simulink model "fixed_point_model"  (R2022b)
settings: Solver=FixedStepDiscrete  StartTime=0.0  StopTime=0.01  FixedStep=1e-10  RelTol=1e-3
undefined symbols (not defined in the file or in its folder): theta_input
libraries: dspsigops x206, dspsrcs4 x16, simulink x8, commdigbbndpm3 x1, commrandsrc3 x1
(part 5 of 6)

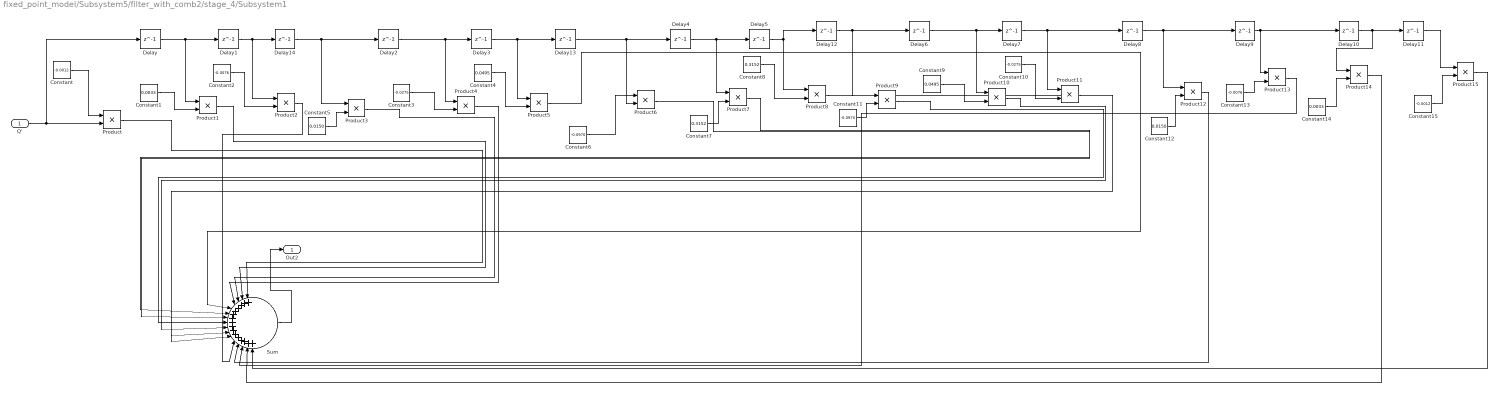
== system fixed_point_model/Subsystem5/filter_with_comb2/stage_4/Subsystem1 ==
  Q' : Inport
  Constant : Constant  Value=-0.0012
  Constant1 : Constant  Value=0.0033
  Constant10 : Constant  Value=-0.0275
  Constant11 : Constant  Value=-0.0970
  Constant12 : Constant  Value=0.0150
  Constant13 : Constant  Value=-0.0076
  Constant14 : Constant  Value=0.0033
  Constant15 : Constant  Value=-0.0012
  Constant2 : Constant  Value=-0.0076
  Constant3 : Constant  Value=-0.0275
  Constant4 : Constant  Value=0.0495
  Constant5 : Constant  Value=0.0150
  Constant6 : Constant  Value=-0.0970
  Constant7 : Constant  Value=0.3152
  Constant8 : Constant  Value=0.3152
  Constant9 : Constant  Value=0.0495
  Delay{,1..14} (15 alike) : Delay  DelayLength=1  InitialCondition=0  InputProcessing=Columns as channels (frame based)
  Product{,1..15} (16 alike) : Product
  Sum : Sum  Inputs=|++++++++++++++++
  Out2 : Outport
  wires:
  Constant1/1 -> Product1/2
  Delay2/1 -> Delay3/1, Product4/1
  Constant10/1 -> Product11/2
  Constant9/1 -> Product10/2
  Delay/1 -> Delay1/1, Product1/1
  Delay4/1 -> Delay5/1, Product7/1
  Constant3/1 -> Product4/2
  Product8/1 -> Sum/11
  Product6/1 -> Sum/6
  Delay1/1 -> Product2/1, Delay14/1
  Delay5/1 -> Delay12/1, Product8/1
  Constant8/1 -> Product8/2
  Q'/1 -> Delay/1, Product/2
  Delay6/1 -> Delay7/1, Product10/1
  Constant/1 -> Product/1
  Constant11/1 -> Product9/2
  Product10/1 -> Sum/9
  Delay7/1 -> Delay8/1, Product11/1
  Product9/1 -> Sum/8
  Delay3/1 -> Product5/1, Delay13/1
  Constant4/1 -> Product5/2
  Product3/1 -> Sum/3
  Product5/1 -> Sum/5
  Constant2/1 -> Product2/2
  Constant5/1 -> Product3/2
  Constant7/1 -> Product7/2
  Product11/1 -> Sum/10
  Constant6/1 -> Product6/1
  Product/1 -> Sum/1
  Product1/1 -> Sum/2
  Product7/1 -> Sum/7
  Product4/1 -> Sum/4
  Sum/1 -> Out2/1
  Product2/1 -> Sum/12
  Constant12/1 -> Product12/2
  Delay8/1 -> Product12/1, Delay9/1
  Constant13/1 -> Product13/2
  Delay9/1 -> Delay10/1, Product13/1
  Constant14/1 -> Product14/2
  Delay10/1 -> Delay11/1, Product14/1
  Delay11/1 -> Product15/1
  Constant15/1 -> Product15/2
  Product12/1 -> Sum/13
  Product13/1 -> Sum/14
  Product14/1 -> Sum/15
  Product15/1 -> Sum/16
  Delay12/1 -> Delay6/1, Product9/1
  Delay13/1 -> Delay4/1, Product6/2
  Delay14/1 -> Delay2/1, Product3/1

== system fixed_point_model/Subsystem6/filter_with_comb1/Stage_1/Subsystem ==
  In1 : Inport
  Constant : Constant
  Constant1 : Constant  Value=42
  Constant2 : Constant  Value=21
  Delay1 : Delay  DelayLength=1  InitialCondition=0  InputProcessing=Columns as channels (frame based)
  Delay2 : Delay  DelayLength=1  InitialCondition=0  InputProcessing=Columns as channels (frame based)
  Product : Product
  Product1 : Product
  Product2 : Product
  Sum : Sum  Inputs=|+++
  Out1 : Outport
  wires:
  Constant1/1 -> Product1/2
  In1/1 -> Product/1, Delay1/1
  Product1/1 -> Sum/2
  Product/1 -> Sum/1
  Sum/1 -> Out1/1
  Constant/1 -> Product/2
  Delay1/1 -> Delay2/1, Product1/1
  Delay2/1 -> Product2/1
  Constant2/1 -> Product2/2
  Product2/1 -> Sum/3

== system fixed_point_model/Subsystem6/filter_with_comb1/Stage_1/Subsystem1 ==
  In2 : Inport
  Constant2 : Constant  Value=3
  Constant3 : Constant  Value=46
  Constant4 : Constant  Value=15
  Delay2 : Delay  DelayLength=1  InitialCondition=0  InputProcessing=Columns as channels (frame based)
  Delay3 : Delay  DelayLength=1  InitialCondition=0  InputProcessing=Columns as channels (frame based)
  Product2 : Product
  Product3 : Product
  Product4 : Product
  Sum1 : Sum  Inputs=|+++
  Out2 : Outport
  wires:
  Delay3/1 -> Product4/1
  Delay2/1 -> Delay3/1, Product3/1
  Sum1/1 -> Out2/1
  Constant2/1 -> Product2/2
  Product2/1 -> Sum1/1
  Constant3/1 -> Product3/2
  Product3/1 -> Sum1/2
  Constant4/1 -> Product4/2
  In2/1 -> Delay2/1, Product2/1
  Product4/1 -> Sum1/3

== system fixed_point_model/Subsystem6/filter_with_comb1/Stage_1/Subsystem2 ==
  In2 : Inport
  Constant2 : Constant  Value=6
  Constant3 : Constant  Value=48
  Constant4 : Constant  Value=10
  Delay2 : Delay  DelayLength=1  InitialCondition=0  InputProcessing=Columns as channels (frame based)
  Delay3 : Delay  DelayLength=1  InitialCondition=0  InputProcessing=Columns as channels (frame based)
  Product2 : Product
  Product3 : Product
  Product4 : Product
  Sum1 : Sum  Inputs=|+++
  Out2 : Outport
  wires:
  In2/1 -> Delay2/1, Product2/1
  Constant4/1 -> Product4/2
  Product2/1 -> Sum1/1
  Constant3/1 -> Product3/2
  Constant2/1 -> Product2/2
  Delay2/1 -> Delay3/1, Product3/1
  Product3/1 -> Sum1/2
  Sum1/1 -> Out2/1
  Delay3/1 -> Product4/1
  Product4/1 -> Sum1/3

== system fixed_point_model/Subsystem6/filter_with_comb1/Stage_1/Subsystem3 ==
  In2 : Inport
  Constant2 : Constant  Value=10
  Constant3 : Constant  Value=48
  Constant4 : Constant  Value=6
  Delay2 : Delay  DelayLength=1  InitialCondition=0  InputProcessing=Columns as channels (frame based)
  Delay3 : Delay  DelayLength=1  InitialCondition=0  InputProcessing=Columns as channels (frame based)
  Product2 : Product
  Product3 : Product
  Product4 : Product
  Sum1 : Sum  Inputs=|+++
  Out2 : Outport
  wires:
  In2/1 -> Delay2/1, Product2/1
  Constant4/1 -> Product4/2
  Product2/1 -> Sum1/1
  Constant3/1 -> Product3/2
  Constant2/1 -> Product2/2
  Delay2/1 -> Delay3/1, Product3/1
  Product3/1 -> Sum1/2
  Sum1/1 -> Out2/1
  Delay3/1 -> Product4/1
  Product4/1 -> Sum1/3

== system fixed_point_model/Subsystem6/filter_with_comb1/Stage_1/Subsystem4 ==
  In2 : Inport
  Constant2 : Constant  Value=15
  Constant3 : Constant  Value=46
  Constant4 : Constant  Value=3
  Delay2 : Delay  DelayLength=1  InitialCondition=0
  Delay3 : Delay  DelayLength=1  InitialCondition=0  InputProcessing=Columns as channels (frame based)
  Product2 : Product
  Product3 : Product
  Product4 : Product
  Sum1 : Sum  Inputs=|+++++
  Out2 : Outport
  wires:
  In2/1 -> Delay2/1, Product2/1
  Product4/1 -> Sum1/4
  Constant4/1 -> Product4/2
  Product2/1 -> Sum1/1
  Constant3/1 -> Product3/2
  Constant2/1 -> Product2/2
  Delay2/1 -> Delay3/1, Product3/1
  Product3/1 -> Sum1/2
  Sum1/1 -> Out2/1
  Delay3/1 -> Product4/1

== system fixed_point_model/Subsystem6/filter_with_comb1/Stage_1/Subsystem5 ==
  In2 : Inport
  Constant2 : Constant  Value=21
  Constant3 : Constant  Value=42
  Constant4 : Constant
  Delay2 : Delay  DelayLength=1  InitialCondition=0  InputProcessing=Columns as channels (frame based)
  Delay3 : Delay  DelayLength=1  InitialCondition=0  InputProcessing=Columns as channels (frame based)
  Product2 : Product
  Product3 : Product
  Product4 : Product
  Sum1 : Sum  Inputs=|+++
  Out2 : Outport
  wires:
  In2/1 -> Delay2/1, Product2/1
  Constant4/1 -> Product4/2
  Product2/1 -> Sum1/1
  Constant3/1 -> Product3/2
  Constant2/1 -> Product2/2
  Delay2/1 -> Delay3/1, Product3/1
  Product3/1 -> Sum1/2
  Sum1/1 -> Out2/1
  Delay3/1 -> Product4/1
  Product4/1 -> Sum1/3

== system fixed_point_model/Subsystem6/filter_with_comb1/Stage_1/Subsystem6 ==
  In2 : Inport
  Constant2 : Constant  Value=28
  Constant3 : Constant  Value=36
  Delay2 : Delay  DelayLength=1  InitialCondition=0  InputProcessing=Columns as channels (frame based)
  Product2 : Product
  Product3 : Product
  Sum1 : Sum  Inputs=|++
  Out2 : Outport
  wires:
  In2/1 -> Delay2/1, Product2/1
  Product2/1 -> Sum1/1
  Constant3/1 -> Product3/2
  Constant2/1 -> Product2/2
  Delay2/1 -> Product3/1
  Product3/1 -> Sum1/2
  Sum1/1 -> Out2/1

== system fixed_point_model/Subsystem6/filter_with_comb1/Stage_1/Subsystem7 ==
  In2 : Inport
  Constant2 : Constant  Value=36
  Constant3 : Constant  Value=28
  Delay2 : Delay  DelayLength=1  InitialCondition=0  InputProcessing=Columns as channels (frame based)
  Product2 : Product
  Product3 : Product
  Sum1 : Sum  Inputs=|++
  Out2 : Outport
  wires:
  In2/1 -> Delay2/1, Product2/1
  Product2/1 -> Sum1/1
  Constant3/1 -> Product3/2
  Constant2/1 -> Product2/2
  Delay2/1 -> Product3/1
  Product3/1 -> Sum1/2
  Sum1/1 -> Out2/1

== system fixed_point_model/Subsystem6/filter_with_comb1/stage_3/Subsystem ==
  In1 : Inport
  Constant : Constant  Value=0.0006
  Constant1 : Constant  Value=-0.0051
  Constant2 : Constant  Value=0.0222
  Constant3 : Constant  Value=-0.0735
  Constant4 : Constant  Value=0.3058
  Constant5 : Constant  Value=0.3058
  Constant6 : Constant  Value=-0.0735
  Constant7 : Constant  Value=0.0222
  Constant8 : Constant  Value=-0.0051
  Constant9 : Constant  Value=0.0006
  Delay{1..9} (9 alike) : Delay  DelayLength=1  InitialCondition=0  InputProcessing=Columns as channels (frame based)
  Product{,1..9} (10 alike) : Product
  Sum : Sum  Inputs=|++++++++++
  Out1 : Outport
  wires:
  Product/1 -> Sum/1
  Product2/1 -> Sum/3
  Delay3/1 -> Product1/1, Delay4/1
  Sum/1 -> Out1/1
  Delay4/1 -> Product2/1, Delay5/1
  Product3/1 -> Sum/4
  In1/1 -> Product/2, Delay3/1
  Constant2/1 -> Product2/2
  Constant3/1 -> Product3/2
  Constant/1 -> Product/1
  Product1/1 -> Sum/2
  Constant1/1 -> Product1/2
  Delay5/1 -> Delay8/1, Product3/1
  Constant7/1 -> Product7/2
  Constant5/1 -> Product5/2
  Constant4/1 -> Product4/1
  Delay6/1 -> Product7/1, Delay9/1
  Delay2/1 -> Delay6/1, Product6/1
  Delay1/1 -> Delay2/1, Product5/1
  Constant6/1 -> Product6/2
  Constant8/1 -> Product8/2
  Constant9/1 -> Product9/2
  Delay7/1 -> Product9/1
  Product5/1 -> Sum/5
  Product6/1 -> Sum/6
  Product7/1 -> Sum/7
  Product8/1 -> Sum/8
  Product9/1 -> Sum/9
  Product4/1 -> Sum/10
  Delay8/1 -> Product4/2, Delay1/1
  Delay9/1 -> Product8/1, Delay7/1

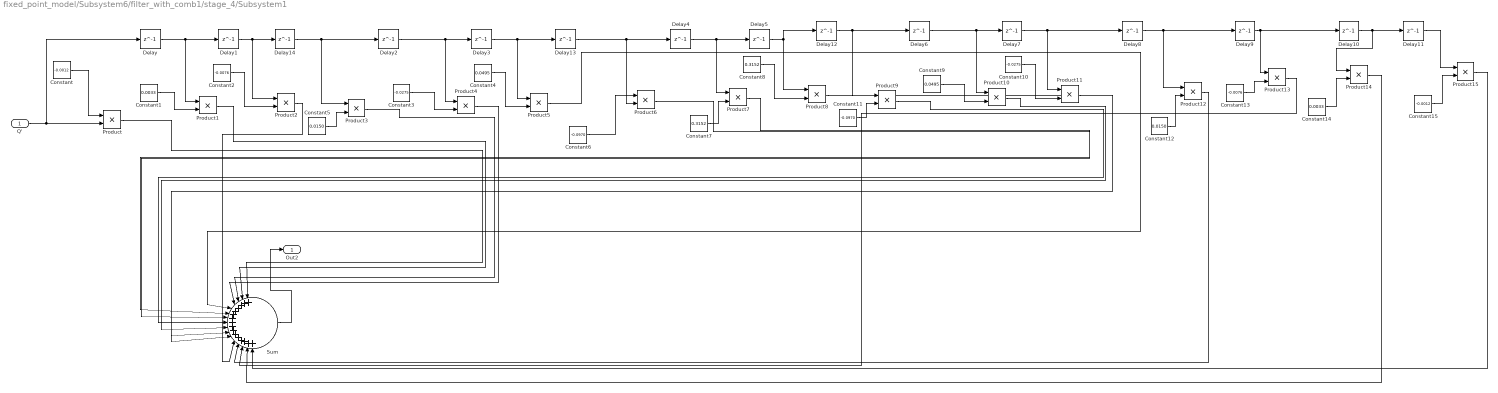
== system fixed_point_model/Subsystem6/filter_with_comb1/stage_4/Subsystem1 ==
  Q' : Inport
  Constant : Constant  Value=-0.0012
  Constant1 : Constant  Value=0.0033
  Constant10 : Constant  Value=-0.0275
  Constant11 : Constant  Value=-0.0970
  Constant12 : Constant  Value=0.0150
  Constant13 : Constant  Value=-0.0076
  Constant14 : Constant  Value=0.0033
  Constant15 : Constant  Value=-0.0012
  Constant2 : Constant  Value=-0.0076
  Constant3 : Constant  Value=-0.0275
  Constant4 : Constant  Value=0.0495
  Constant5 : Constant  Value=0.0150
  Constant6 : Constant  Value=-0.0970
  Constant7 : Constant  Value=0.3152
  Constant8 : Constant  Value=0.3152
  Constant9 : Constant  Value=0.0495
  Delay{,1..14} (15 alike) : Delay  DelayLength=1  InitialCondition=0  InputProcessing=Columns as channels (frame based)
  Product{,1..15} (16 alike) : Product
  Sum : Sum  Inputs=|++++++++++++++++
  Out2 : Outport
  wires:
  Constant1/1 -> Product1/2
  Delay2/1 -> Delay3/1, Product4/1
  Constant10/1 -> Product11/2
  Constant9/1 -> Product10/2
  Delay/1 -> Delay1/1, Product1/1
  Delay4/1 -> Delay5/1, Product7/1
  Constant3/1 -> Product4/2
  Product8/1 -> Sum/11
  Product6/1 -> Sum/6
  Delay1/1 -> Product2/1, Delay14/1
  Delay5/1 -> Delay12/1, Product8/1
  Constant8/1 -> Product8/2
  Q'/1 -> Delay/1, Product/2
  Delay6/1 -> Delay7/1, Product10/1
  Constant/1 -> Product/1
  Constant11/1 -> Product9/2
  Product10/1 -> Sum/9
  Delay7/1 -> Delay8/1, Product11/1
  Product9/1 -> Sum/8
  Delay3/1 -> Product5/1, Delay13/1
  Constant4/1 -> Product5/2
  Product3/1 -> Sum/3
  Product5/1 -> Sum/5
  Constant2/1 -> Product2/2
  Constant5/1 -> Product3/2
  Constant7/1 -> Product7/2
  Product11/1 -> Sum/10
  Constant6/1 -> Product6/1
  Product/1 -> Sum/1
  Product1/1 -> Sum/2
  Product7/1 -> Sum/7
  Product4/1 -> Sum/4
  Sum/1 -> Out2/1
  Product2/1 -> Sum/12
  Constant12/1 -> Product12/2
  Delay8/1 -> Product12/1, Delay9/1
  Constant13/1 -> Product13/2
  Delay9/1 -> Delay10/1, Product13/1
  Constant14/1 -> Product14/2
  Delay10/1 -> Delay11/1, Product14/1
  Delay11/1 -> Product15/1
  Constant15/1 -> Product15/2
  Product12/1 -> Sum/13
  Product13/1 -> Sum/14
  Product14/1 -> Sum/15
  Product15/1 -> Sum/16
  Delay12/1 -> Delay6/1, Product9/1
  Delay13/1 -> Delay4/1, Product6/2
  Delay14/1 -> Delay2/1, Product3/1

== system fixed_point_model/Subsystem6/filter_with_comb2/Stage_1/Subsystem ==
  In1 : Inport
  Constant : Constant
  Constant1 : Constant  Value=42
  Constant2 : Constant  Value=21
  Delay1 : Delay  DelayLength=1  InitialCondition=0  InputProcessing=Columns as channels (frame based)
  Delay2 : Delay  DelayLength=1  InitialCondition=0  InputProcessing=Columns as channels (frame based)
  Product : Product
  Product1 : Product
  Product2 : Product
  Sum : Sum  Inputs=|+++
  Out1 : Outport
  wires:
  Constant1/1 -> Product1/2
  In1/1 -> Product/1, Delay1/1
  Product1/1 -> Sum/2
  Product/1 -> Sum/1
  Sum/1 -> Out1/1
  Constant/1 -> Product/2
  Delay1/1 -> Delay2/1, Product1/1
  Delay2/1 -> Product2/1
  Constant2/1 -> Product2/2
  Product2/1 -> Sum/3

== system fixed_point_model/Subsystem6/filter_with_comb2/Stage_1/Subsystem1 ==
  In2 : Inport
  Constant2 : Constant  Value=3
  Constant3 : Constant  Value=46
  Constant4 : Constant  Value=15
  Delay2 : Delay  DelayLength=1  InitialCondition=0  InputProcessing=Columns as channels (frame based)
  Delay3 : Delay  DelayLength=1  InitialCondition=0  InputProcessing=Columns as channels (frame based)
  Product2 : Product
  Product3 : Product
  Product4 : Product
  Sum1 : Sum  Inputs=|+++
  Out2 : Outport
  wires:
  Delay3/1 -> Product4/1
  Delay2/1 -> Delay3/1, Product3/1
  Sum1/1 -> Out2/1
  Constant2/1 -> Product2/2
  Product2/1 -> Sum1/1
  Constant3/1 -> Product3/2
  Product3/1 -> Sum1/2
  Constant4/1 -> Product4/2
  In2/1 -> Delay2/1, Product2/1
  Product4/1 -> Sum1/3

== system fixed_point_model/Subsystem6/filter_with_comb2/Stage_1/Subsystem2 ==
  In2 : Inport
  Constant2 : Constant  Value=6
  Constant3 : Constant  Value=48
  Constant4 : Constant  Value=10
  Delay2 : Delay  DelayLength=1  InitialCondition=0  InputProcessing=Columns as channels (frame based)
  Delay3 : Delay  DelayLength=1  InitialCondition=0  InputProcessing=Columns as channels (frame based)
  Product2 : Product
  Product3 : Product
  Product4 : Product
  Sum1 : Sum  Inputs=|+++
  Out2 : Outport
  wires:
  In2/1 -> Delay2/1, Product2/1
  Constant4/1 -> Product4/2
  Product2/1 -> Sum1/1
  Constant3/1 -> Product3/2
  Constant2/1 -> Product2/2
  Delay2/1 -> Delay3/1, Product3/1
  Product3/1 -> Sum1/2
  Sum1/1 -> Out2/1
  Delay3/1 -> Product4/1
  Product4/1 -> Sum1/3

== system fixed_point_model/Subsystem6/filter_with_comb2/Stage_1/Subsystem3 ==
  In2 : Inport
  Constant2 : Constant  Value=10
  Constant3 : Constant  Value=48
  Constant4 : Constant  Value=6
  Delay2 : Delay  DelayLength=1  InitialCondition=0  InputProcessing=Columns as channels (frame based)
  Delay3 : Delay  DelayLength=1  InitialCondition=0  InputProcessing=Columns as channels (frame based)
  Product2 : Product
  Product3 : Product
  Product4 : Product
  Sum1 : Sum  Inputs=|+++
  Out2 : Outport
  wires:
  In2/1 -> Delay2/1, Product2/1
  Constant4/1 -> Product4/2
  Product2/1 -> Sum1/1
  Constant3/1 -> Product3/2
  Constant2/1 -> Product2/2
  Delay2/1 -> Delay3/1, Product3/1
  Product3/1 -> Sum1/2
  Sum1/1 -> Out2/1
  Delay3/1 -> Product4/1
  Product4/1 -> Sum1/3

== system fixed_point_model/Subsystem6/filter_with_comb2/Stage_1/Subsystem4 ==
  In2 : Inport
  Constant2 : Constant  Value=15
  Constant3 : Constant  Value=46
  Constant4 : Constant  Value=3
  Delay2 : Delay  DelayLength=1  InitialCondition=0
  Delay3 : Delay  DelayLength=1  InitialCondition=0  InputProcessing=Columns as channels (frame based)
  Product2 : Product
  Product3 : Product
  Product4 : Product
  Sum1 : Sum  Inputs=|+++++
  Out2 : Outport
  wires:
  In2/1 -> Delay2/1, Product2/1
  Product4/1 -> Sum1/4
  Constant4/1 -> Product4/2
  Product2/1 -> Sum1/1
  Constant3/1 -> Product3/2
  Constant2/1 -> Product2/2
  Delay2/1 -> Delay3/1, Product3/1
  Product3/1 -> Sum1/2
  Sum1/1 -> Out2/1
  Delay3/1 -> Product4/1

== system fixed_point_model/Subsystem6/filter_with_comb2/Stage_1/Subsystem5 ==
  In2 : Inport
  Constant2 : Constant  Value=21
  Constant3 : Constant  Value=42
  Constant4 : Constant
  Delay2 : Delay  DelayLength=1  InitialCondition=0  InputProcessing=Columns as channels (frame based)
  Delay3 : Delay  DelayLength=1  InitialCondition=0  InputProcessing=Columns as channels (frame based)
  Product2 : Product
  Product3 : Product
  Product4 : Product
  Sum1 : Sum  Inputs=|+++
  Out2 : Outport
  wires:
  In2/1 -> Delay2/1, Product2/1
  Constant4/1 -> Product4/2
  Product2/1 -> Sum1/1
  Constant3/1 -> Product3/2
  Constant2/1 -> Product2/2
  Delay2/1 -> Delay3/1, Product3/1
  Product3/1 -> Sum1/2
  Sum1/1 -> Out2/1
  Delay3/1 -> Product4/1
  Product4/1 -> Sum1/3

== system fixed_point_model/Subsystem6/filter_with_comb2/Stage_1/Subsystem6 ==
  In2 : Inport
  Constant2 : Constant  Value=28
  Constant3 : Constant  Value=36
  Delay2 : Delay  DelayLength=1  InitialCondition=0  InputProcessing=Columns as channels (frame based)
  Product2 : Product
  Product3 : Product
  Sum1 : Sum  Inputs=|++
  Out2 : Outport
  wires:
  In2/1 -> Delay2/1, Product2/1
  Product2/1 -> Sum1/1
  Constant3/1 -> Product3/2
  Constant2/1 -> Product2/2
  Delay2/1 -> Product3/1
  Product3/1 -> Sum1/2
  Sum1/1 -> Out2/1

== system fixed_point_model/Subsystem6/filter_with_comb2/Stage_1/Subsystem7 ==
  In2 : Inport
  Constant2 : Constant  Value=36
  Constant3 : Constant  Value=28
  Delay2 : Delay  DelayLength=1  InitialCondition=0  InputProcessing=Columns as channels (frame based)
  Product2 : Product
  Product3 : Product
  Sum1 : Sum  Inputs=|++
  Out2 : Outport
  wires:
  In2/1 -> Delay2/1, Product2/1
  Product2/1 -> Sum1/1
  Constant3/1 -> Product3/2
  Constant2/1 -> Product2/2
  Delay2/1 -> Product3/1
  Product3/1 -> Sum1/2
  Sum1/1 -> Out2/1

== system fixed_point_model/Subsystem6/filter_with_comb2/stage_3/Subsystem ==
  In1 : Inport
  Constant : Constant  Value=0.0006
  Constant1 : Constant  Value=-0.0051
  Constant2 : Constant  Value=0.0222
  Constant3 : Constant  Value=-0.0735
  Constant4 : Constant  Value=0.3058
  Constant5 : Constant  Value=0.3058
  Constant6 : Constant  Value=-0.0735
  Constant7 : Constant  Value=0.0222
  Constant8 : Constant  Value=-0.0051
  Constant9 : Constant  Value=0.0006
  Delay{1..9} (9 alike) : Delay  DelayLength=1  InitialCondition=0  InputProcessing=Columns as channels (frame based)
  Product{,1..9} (10 alike) : Product
  Sum : Sum  Inputs=|++++++++++
  Out1 : Outport
  wires:
  Product/1 -> Sum/1
  Product2/1 -> Sum/3
  Delay3/1 -> Product1/1, Delay4/1
  Sum/1 -> Out1/1
  Delay4/1 -> Product2/1, Delay5/1
  Product3/1 -> Sum/4
  In1/1 -> Product/2, Delay3/1
  Constant2/1 -> Product2/2
  Constant3/1 -> Product3/2
  Constant/1 -> Product/1
  Product1/1 -> Sum/2
  Constant1/1 -> Product1/2
  Delay5/1 -> Delay8/1, Product3/1
  Constant7/1 -> Product7/2
  Constant5/1 -> Product5/2
  Constant4/1 -> Product4/1
  Delay6/1 -> Product7/1, Delay9/1
  Delay2/1 -> Delay6/1, Product6/1
  Delay1/1 -> Delay2/1, Product5/1
  Constant6/1 -> Product6/2
  Constant8/1 -> Product8/2
  Constant9/1 -> Product9/2
  Delay7/1 -> Product9/1
  Product5/1 -> Sum/5
  Product6/1 -> Sum/6
  Product7/1 -> Sum/7
  Product8/1 -> Sum/8
  Product9/1 -> Sum/9
  Product4/1 -> Sum/10
  Delay8/1 -> Product4/2, Delay1/1
  Delay9/1 -> Product8/1, Delay7/1

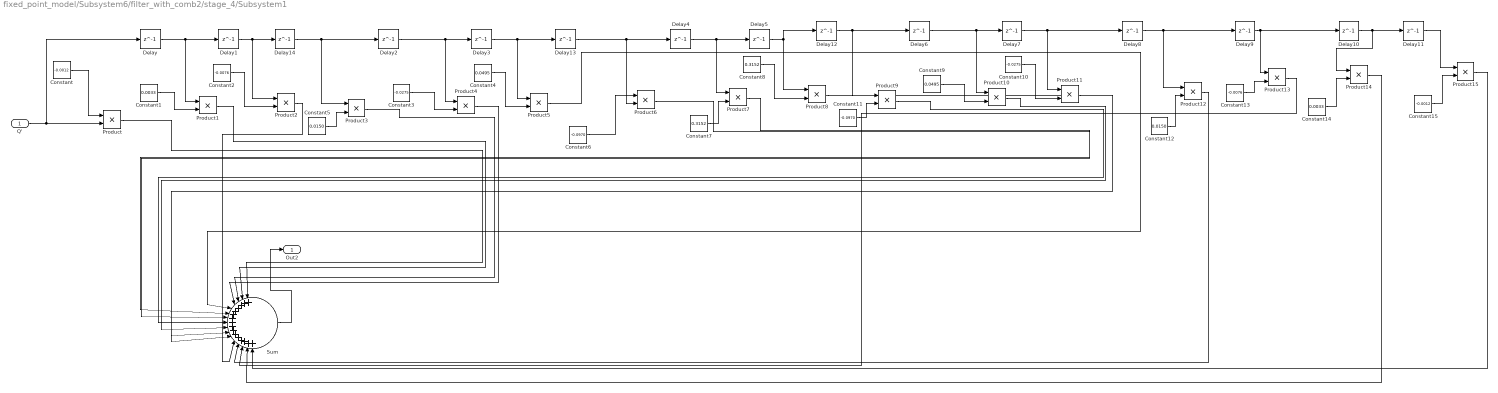
== system fixed_point_model/Subsystem6/filter_with_comb2/stage_4/Subsystem1 ==
  Q' : Inport
  Constant : Constant  Value=-0.0012
  Constant1 : Constant  Value=0.0033
  Constant10 : Constant  Value=-0.0275
  Constant11 : Constant  Value=-0.0970
  Constant12 : Constant  Value=0.0150
  Constant13 : Constant  Value=-0.0076
  Constant14 : Constant  Value=0.0033
  Constant15 : Constant  Value=-0.0012
  Constant2 : Constant  Value=-0.0076
  Constant3 : Constant  Value=-0.0275
  Constant4 : Constant  Value=0.0495
  Constant5 : Constant  Value=0.0150
  Constant6 : Constant  Value=-0.0970
  Constant7 : Constant  Value=0.3152
  Constant8 : Constant  Value=0.3152
  Constant9 : Constant  Value=0.0495
  Delay{,1..14} (15 alike) : Delay  DelayLength=1  InitialCondition=0  InputProcessing=Columns as channels (frame based)
  Product{,1..15} (16 alike) : Product
  Sum : Sum  Inputs=|++++++++++++++++
  Out2 : Outport
  wires:
  Constant1/1 -> Product1/2
  Delay2/1 -> Delay3/1, Product4/1
  Constant10/1 -> Product11/2
  Constant9/1 -> Product10/2
  Delay/1 -> Delay1/1, Product1/1
  Delay4/1 -> Delay5/1, Product7/1
  Constant3/1 -> Product4/2
  Product8/1 -> Sum/11
  Product6/1 -> Sum/6
  Delay1/1 -> Product2/1, Delay14/1
  Delay5/1 -> Delay12/1, Product8/1
  Constant8/1 -> Product8/2
  Q'/1 -> Delay/1, Product/2
  Delay6/1 -> Delay7/1, Product10/1
  Constant/1 -> Product/1
  Constant11/1 -> Product9/2
  Product10/1 -> Sum/9
  Delay7/1 -> Delay8/1, Product11/1
  Product9/1 -> Sum/8
  Delay3/1 -> Product5/1, Delay13/1
  Constant4/1 -> Product5/2
  Product3/1 -> Sum/3
  Product5/1 -> Sum/5
  Constant2/1 -> Product2/2
  Constant5/1 -> Product3/2
  Constant7/1 -> Product7/2
  Product11/1 -> Sum/10
  Constant6/1 -> Product6/1
  Product/1 -> Sum/1
  Product1/1 -> Sum/2
  Product7/1 -> Sum/7
  Product4/1 -> Sum/4
  Sum/1 -> Out2/1
  Product2/1 -> Sum/12
  Constant12/1 -> Product12/2
  Delay8/1 -> Product12/1, Delay9/1
  Constant13/1 -> Product13/2
  Delay9/1 -> Delay10/1, Product13/1
  Constant14/1 -> Product14/2
  Delay10/1 -> Delay11/1, Product14/1
  Delay11/1 -> Product15/1
  Constant15/1 -> Product15/2
  Product12/1 -> Sum/13
  Product13/1 -> Sum/14
  Product14/1 -> Sum/15
  Product15/1 -> Sum/16
  Delay12/1 -> Delay6/1, Product9/1
  Delay13/1 -> Delay4/1, Product6/2
  Delay14/1 -> Delay2/1, Product3/1

== system fixed_point_model/Subsystem7/filter_with_comb1/Stage_1/Subsystem ==
  In1 : Inport
  Constant : Constant
  Constant1 : Constant  Value=42
  Constant2 : Constant  Value=21
  Delay1 : Delay  DelayLength=1  InitialCondition=0  InputProcessing=Columns as channels (frame based)
  Delay2 : Delay  DelayLength=1  InitialCondition=0  InputProcessing=Columns as channels (frame based)
  Product : Product
  Product1 : Product
  Product2 : Product
  Sum : Sum  Inputs=|+++
  Out1 : Outport
  wires:
  Constant1/1 -> Product1/2
  In1/1 -> Product/1, Delay1/1
  Product1/1 -> Sum/2
  Product/1 -> Sum/1
  Sum/1 -> Out1/1
  Constant/1 -> Product/2
  Delay1/1 -> Delay2/1, Product1/1
  Delay2/1 -> Product2/1
  Constant2/1 -> Product2/2
  Product2/1 -> Sum/3

== system fixed_point_model/Subsystem7/filter_with_comb1/Stage_1/Subsystem1 ==
  In2 : Inport
  Constant2 : Constant  Value=3
  Constant3 : Constant  Value=46
  Constant4 : Constant  Value=15
  Delay2 : Delay  DelayLength=1  InitialCondition=0  InputProcessing=Columns as channels (frame based)
  Delay3 : Delay  DelayLength=1  InitialCondition=0  InputProcessing=Columns as channels (frame based)
  Product2 : Product
  Product3 : Product
  Product4 : Product
  Sum1 : Sum  Inputs=|+++
  Out2 : Outport
  wires:
  Delay3/1 -> Product4/1
  Delay2/1 -> Delay3/1, Product3/1
  Sum1/1 -> Out2/1
  Constant2/1 -> Product2/2
  Product2/1 -> Sum1/1
  Constant3/1 -> Product3/2
  Product3/1 -> Sum1/2
  Constant4/1 -> Product4/2
  In2/1 -> Delay2/1, Product2/1
  Product4/1 -> Sum1/3

== system fixed_point_model/Subsystem7/filter_with_comb1/Stage_1/Subsystem2 ==
  In2 : Inport
  Constant2 : Constant  Value=6
  Constant3 : Constant  Value=48
  Constant4 : Constant  Value=10
  Delay2 : Delay  DelayLength=1  InitialCondition=0  InputProcessing=Columns as channels (frame based)
  Delay3 : Delay  DelayLength=1  InitialCondition=0  InputProcessing=Columns as channels (frame based)
  Product2 : Product
  Product3 : Product
  Product4 : Product
  Sum1 : Sum  Inputs=|+++
  Out2 : Outport
  wires:
  In2/1 -> Delay2/1, Product2/1
  Constant4/1 -> Product4/2
  Product2/1 -> Sum1/1
  Constant3/1 -> Product3/2
  Constant2/1 -> Product2/2
  Delay2/1 -> Delay3/1, Product3/1
  Product3/1 -> Sum1/2
  Sum1/1 -> Out2/1
  Delay3/1 -> Product4/1
  Product4/1 -> Sum1/3

== system fixed_point_model/Subsystem7/filter_with_comb1/Stage_1/Subsystem3 ==
  In2 : Inport
  Constant2 : Constant  Value=10
  Constant3 : Constant  Value=48
  Constant4 : Constant  Value=6
  Delay2 : Delay  DelayLength=1  InitialCondition=0  InputProcessing=Columns as channels (frame based)
  Delay3 : Delay  DelayLength=1  InitialCondition=0  InputProcessing=Columns as channels (frame based)
  Product2 : Product
  Product3 : Product
  Product4 : Product
  Sum1 : Sum  Inputs=|+++
  Out2 : Outport
  wires:
  In2/1 -> Delay2/1, Product2/1
  Constant4/1 -> Product4/2
  Product2/1 -> Sum1/1
  Constant3/1 -> Product3/2
  Constant2/1 -> Product2/2
  Delay2/1 -> Delay3/1, Product3/1
  Product3/1 -> Sum1/2
  Sum1/1 -> Out2/1
  Delay3/1 -> Product4/1
  Product4/1 -> Sum1/3

== system fixed_point_model/Subsystem7/filter_with_comb1/Stage_1/Subsystem4 ==
  In2 : Inport
  Constant2 : Constant  Value=15
  Constant3 : Constant  Value=46
  Constant4 : Constant  Value=3
  Delay2 : Delay  DelayLength=1  InitialCondition=0
  Delay3 : Delay  DelayLength=1  InitialCondition=0  InputProcessing=Columns as channels (frame based)
  Product2 : Product
  Product3 : Product
  Product4 : Product
  Sum1 : Sum  Inputs=|+++++
  Out2 : Outport
  wires:
  In2/1 -> Delay2/1, Product2/1
  Product4/1 -> Sum1/4
  Constant4/1 -> Product4/2
  Product2/1 -> Sum1/1
  Constant3/1 -> Product3/2
  Constant2/1 -> Product2/2
  Delay2/1 -> Delay3/1, Product3/1
  Product3/1 -> Sum1/2
  Sum1/1 -> Out2/1
  Delay3/1 -> Product4/1

== system fixed_point_model/Subsystem7/filter_with_comb1/Stage_1/Subsystem5 ==
  In2 : Inport
  Constant2 : Constant  Value=21
  Constant3 : Constant  Value=42
  Constant4 : Constant
  Delay2 : Delay  DelayLength=1  InitialCondition=0  InputProcessing=Columns as channels (frame based)
  Delay3 : Delay  DelayLength=1  InitialCondition=0  InputProcessing=Columns as channels (frame based)
  Product2 : Product
  Product3 : Product
  Product4 : Product
  Sum1 : Sum  Inputs=|+++
  Out2 : Outport
  wires:
  In2/1 -> Delay2/1, Product2/1
  Constant4/1 -> Product4/2
  Product2/1 -> Sum1/1
  Constant3/1 -> Product3/2
  Constant2/1 -> Product2/2
  Delay2/1 -> Delay3/1, Product3/1
  Product3/1 -> Sum1/2
  Sum1/1 -> Out2/1
  Delay3/1 -> Product4/1
  Product4/1 -> Sum1/3

== system fixed_point_model/Subsystem7/filter_with_comb1/Stage_1/Subsystem6 ==
  In2 : Inport
  Constant2 : Constant  Value=28
  Constant3 : Constant  Value=36
  Delay2 : Delay  DelayLength=1  InitialCondition=0  InputProcessing=Columns as channels (frame based)
  Product2 : Product
  Product3 : Product
  Sum1 : Sum  Inputs=|++
  Out2 : Outport
  wires:
  In2/1 -> Delay2/1, Product2/1
  Product2/1 -> Sum1/1
  Constant3/1 -> Product3/2
  Constant2/1 -> Product2/2
  Delay2/1 -> Product3/1
  Product3/1 -> Sum1/2
  Sum1/1 -> Out2/1

== system fixed_point_model/Subsystem7/filter_with_comb1/Stage_1/Subsystem7 ==
  In2 : Inport
  Constant2 : Constant  Value=36
  Constant3 : Constant  Value=28
  Delay2 : Delay  DelayLength=1  InitialCondition=0  InputProcessing=Columns as channels (frame based)
  Product2 : Product
  Product3 : Product
  Sum1 : Sum  Inputs=|++
  Out2 : Outport
  wires:
  In2/1 -> Delay2/1, Product2/1
  Product2/1 -> Sum1/1
  Constant3/1 -> Product3/2
  Constant2/1 -> Product2/2
  Delay2/1 -> Product3/1
  Product3/1 -> Sum1/2
  Sum1/1 -> Out2/1

== system fixed_point_model/Subsystem7/filter_with_comb1/stage_3/Subsystem ==
  In1 : Inport
  Constant : Constant  Value=0.0006
  Constant1 : Constant  Value=-0.0051
  Constant2 : Constant  Value=0.0222
  Constant3 : Constant  Value=-0.0735
  Constant4 : Constant  Value=0.3058
  Constant5 : Constant  Value=0.3058
  Constant6 : Constant  Value=-0.0735
  Constant7 : Constant  Value=0.0222
  Constant8 : Constant  Value=-0.0051
  Constant9 : Constant  Value=0.0006
  Delay{1..9} (9 alike) : Delay  DelayLength=1  InitialCondition=0  InputProcessing=Columns as channels (frame based)
  Product{,1..9} (10 alike) : Product
  Sum : Sum  Inputs=|++++++++++
  Out1 : Outport
  wires:
  Product/1 -> Sum/1
  Product2/1 -> Sum/3
  Delay3/1 -> Product1/1, Delay4/1
  Sum/1 -> Out1/1
  Delay4/1 -> Product2/1, Delay5/1
  Product3/1 -> Sum/4
  In1/1 -> Product/2, Delay3/1
  Constant2/1 -> Product2/2
  Constant3/1 -> Product3/2
  Constant/1 -> Product/1
  Product1/1 -> Sum/2
  Constant1/1 -> Product1/2
  Delay5/1 -> Delay8/1, Product3/1
  Constant7/1 -> Product7/2
  Constant5/1 -> Product5/2
  Constant4/1 -> Product4/1
  Delay6/1 -> Product7/1, Delay9/1
  Delay2/1 -> Delay6/1, Product6/1
  Delay1/1 -> Delay2/1, Product5/1
  Constant6/1 -> Product6/2
  Constant8/1 -> Product8/2
  Constant9/1 -> Product9/2
  Delay7/1 -> Product9/1
  Product5/1 -> Sum/5
  Product6/1 -> Sum/6
  Product7/1 -> Sum/7
  Product8/1 -> Sum/8
  Product9/1 -> Sum/9
  Product4/1 -> Sum/10
  Delay8/1 -> Product4/2, Delay1/1
  Delay9/1 -> Product8/1, Delay7/1

== system fixed_point_model/Subsystem7/filter_with_comb1/stage_4/Subsystem1 ==
  Q' : Inport
  Constant : Constant  Value=-0.0012
  Constant1 : Constant  Value=0.0033
  Constant10 : Constant  Value=-0.0275
  Constant11 : Constant  Value=-0.0970
  Constant12 : Constant  Value=0.0150
  Constant13 : Constant  Value=-0.0076
  Constant14 : Constant  Value=0.0033
  Constant15 : Constant  Value=-0.0012
  Constant2 : Constant  Value=-0.0076
  Constant3 : Constant  Value=-0.0275
  Constant4 : Constant  Value=0.0495
  Constant5 : Constant  Value=0.0150
  Constant6 : Constant  Value=-0.0970
  Constant7 : Constant  Value=0.3152
  Constant8 : Constant  Value=0.3152
  Constant9 : Constant  Value=0.0495
  Delay{,1..14} (15 alike) : Delay  DelayLength=1  InitialCondition=0  InputProcessing=Columns as channels (frame based)
  Product{,1..15} (16 alike) : Product
  Sum : Sum  Inputs=|++++++++++++++++
  Out2 : Outport
  wires:
  Constant1/1 -> Product1/2
  Delay2/1 -> Delay3/1, Product4/1
  Constant10/1 -> Product11/2
  Constant9/1 -> Product10/2
  Delay/1 -> Delay1/1, Product1/1
  Delay4/1 -> Delay5/1, Product7/1
  Constant3/1 -> Product4/2
  Product8/1 -> Sum/11
  Product6/1 -> Sum/6
  Delay1/1 -> Product2/1, Delay14/1
  Delay5/1 -> Delay12/1, Product8/1
  Constant8/1 -> Product8/2
  Q'/1 -> Delay/1, Product/2
  Delay6/1 -> Delay7/1, Product10/1
  Constant/1 -> Product/1
  Constant11/1 -> Product9/2
  Product10/1 -> Sum/9
  Delay7/1 -> Delay8/1, Product11/1
  Product9/1 -> Sum/8
  Delay3/1 -> Product5/1, Delay13/1
  Constant4/1 -> Product5/2
  Product3/1 -> Sum/3
  Product5/1 -> Sum/5
  Constant2/1 -> Product2/2
  Constant5/1 -> Product3/2
  Constant7/1 -> Product7/2
  Product11/1 -> Sum/10
  Constant6/1 -> Product6/1
  Product/1 -> Sum/1
  Product1/1 -> Sum/2
  Product7/1 -> Sum/7
  Product4/1 -> Sum/4
  Sum/1 -> Out2/1
  Product2/1 -> Sum/12
  Constant12/1 -> Product12/2
  Delay8/1 -> Product12/1, Delay9/1
  Constant13/1 -> Product13/2
  Delay9/1 -> Delay10/1, Product13/1
  Constant14/1 -> Product14/2
  Delay10/1 -> Delay11/1, Product14/1
  Delay11/1 -> Product15/1
  Constant15/1 -> Product15/2
  Product12/1 -> Sum/13
  Product13/1 -> Sum/14
  Product14/1 -> Sum/15
  Product15/1 -> Sum/16
  Delay12/1 -> Delay6/1, Product9/1
  Delay13/1 -> Delay4/1, Product6/2
  Delay14/1 -> Delay2/1, Product3/1

== system fixed_point_model/Subsystem7/filter_with_comb2/Stage_1/Subsystem ==
  In1 : Inport
  Constant : Constant
  Constant1 : Constant  Value=42
  Constant2 : Constant  Value=21
  Delay1 : Delay  DelayLength=1  InitialCondition=0  InputProcessing=Columns as channels (frame based)
  Delay2 : Delay  DelayLength=1  InitialCondition=0  InputProcessing=Columns as channels (frame based)
  Product : Product
  Product1 : Product
  Product2 : Product
  Sum : Sum  Inputs=|+++
  Out1 : Outport
  wires:
  Constant1/1 -> Product1/2
  In1/1 -> Product/1, Delay1/1
  Product1/1 -> Sum/2
  Product/1 -> Sum/1
  Sum/1 -> Out1/1
  Constant/1 -> Product/2
  Delay1/1 -> Delay2/1, Product1/1
  Delay2/1 -> Product2/1
  Constant2/1 -> Product2/2
  Product2/1 -> Sum/3

== system fixed_point_model/Subsystem7/filter_with_comb2/Stage_1/Subsystem1 ==
  In2 : Inport
  Constant2 : Constant  Value=3
  Constant3 : Constant  Value=46
  Constant4 : Constant  Value=15
  Delay2 : Delay  DelayLength=1  InitialCondition=0  InputProcessing=Columns as channels (frame based)
  Delay3 : Delay  DelayLength=1  InitialCondition=0  InputProcessing=Columns as channels (frame based)
  Product2 : Product
  Product3 : Product
  Product4 : Product
  Sum1 : Sum  Inputs=|+++
  Out2 : Outport
  wires:
  Delay3/1 -> Product4/1
  Delay2/1 -> Delay3/1, Product3/1
  Sum1/1 -> Out2/1
  Constant2/1 -> Product2/2
  Product2/1 -> Sum1/1
  Constant3/1 -> Product3/2
  Product3/1 -> Sum1/2
  Constant4/1 -> Product4/2
  In2/1 -> Delay2/1, Product2/1
  Product4/1 -> Sum1/3

== system fixed_point_model/Subsystem7/filter_with_comb2/Stage_1/Subsystem2 ==
  In2 : Inport
  Constant2 : Constant  Value=6
  Constant3 : Constant  Value=48
  Constant4 : Constant  Value=10
  Delay2 : Delay  DelayLength=1  InitialCondition=0  InputProcessing=Columns as channels (frame based)
  Delay3 : Delay  DelayLength=1  InitialCondition=0  InputProcessing=Columns as channels (frame based)
  Product2 : Product
  Product3 : Product
  Product4 : Product
  Sum1 : Sum  Inputs=|+++
  Out2 : Outport
  wires:
  In2/1 -> Delay2/1, Product2/1
  Constant4/1 -> Product4/2
  Product2/1 -> Sum1/1
  Constant3/1 -> Product3/2
  Constant2/1 -> Product2/2
  Delay2/1 -> Delay3/1, Product3/1
  Product3/1 -> Sum1/2
  Sum1/1 -> Out2/1
  Delay3/1 -> Product4/1
  Product4/1 -> Sum1/3

== system fixed_point_model/Subsystem7/filter_with_comb2/Stage_1/Subsystem3 ==
  In2 : Inport
  Constant2 : Constant  Value=10
  Constant3 : Constant  Value=48
  Constant4 : Constant  Value=6
  Delay2 : Delay  DelayLength=1  InitialCondition=0  InputProcessing=Columns as channels (frame based)
  Delay3 : Delay  DelayLength=1  InitialCondition=0  InputProcessing=Columns as channels (frame based)
  Product2 : Product
  Product3 : Product
  Product4 : Product
  Sum1 : Sum  Inputs=|+++
  Out2 : Outport
  wires:
  In2/1 -> Delay2/1, Product2/1
  Constant4/1 -> Product4/2
  Product2/1 -> Sum1/1
  Constant3/1 -> Product3/2
  Constant2/1 -> Product2/2
  Delay2/1 -> Delay3/1, Product3/1
  Product3/1 -> Sum1/2
  Sum1/1 -> Out2/1
  Delay3/1 -> Product4/1
  Product4/1 -> Sum1/3

== system fixed_point_model/Subsystem7/filter_with_comb2/Stage_1/Subsystem4 ==
  In2 : Inport
  Constant2 : Constant  Value=15
  Constant3 : Constant  Value=46
  Constant4 : Constant  Value=3
  Delay2 : Delay  DelayLength=1  InitialCondition=0
  Delay3 : Delay  DelayLength=1  InitialCondition=0  InputProcessing=Columns as channels (frame based)
  Product2 : Product
  Product3 : Product
  Product4 : Product
  Sum1 : Sum  Inputs=|+++++
  Out2 : Outport
  wires:
  In2/1 -> Delay2/1, Product2/1
  Product4/1 -> Sum1/4
  Constant4/1 -> Product4/2
  Product2/1 -> Sum1/1
  Constant3/1 -> Product3/2
  Constant2/1 -> Product2/2
  Delay2/1 -> Delay3/1, Product3/1
  Product3/1 -> Sum1/2
  Sum1/1 -> Out2/1
  Delay3/1 -> Product4/1

== system fixed_point_model/Subsystem7/filter_with_comb2/Stage_1/Subsystem5 ==
  In2 : Inport
  Constant2 : Constant  Value=21
  Constant3 : Constant  Value=42
  Constant4 : Constant
  Delay2 : Delay  DelayLength=1  InitialCondition=0  InputProcessing=Columns as channels (frame based)
  Delay3 : Delay  DelayLength=1  InitialCondition=0  InputProcessing=Columns as channels (frame based)
  Product2 : Product
  Product3 : Product
  Product4 : Product
  Sum1 : Sum  Inputs=|+++
  Out2 : Outport
  wires:
  In2/1 -> Delay2/1, Product2/1
  Constant4/1 -> Product4/2
  Product2/1 -> Sum1/1
  Constant3/1 -> Product3/2
  Constant2/1 -> Product2/2
  Delay2/1 -> Delay3/1, Product3/1
  Product3/1 -> Sum1/2
  Sum1/1 -> Out2/1
  Delay3/1 -> Product4/1
  Product4/1 -> Sum1/3

== system fixed_point_model/Subsystem7/filter_with_comb2/Stage_1/Subsystem6 ==
  In2 : Inport
  Constant2 : Constant  Value=28
  Constant3 : Constant  Value=36
  Delay2 : Delay  DelayLength=1  InitialCondition=0  InputProcessing=Columns as channels (frame based)
  Product2 : Product
  Product3 : Product
  Sum1 : Sum  Inputs=|++
  Out2 : Outport
  wires:
  In2/1 -> Delay2/1, Product2/1
  Product2/1 -> Sum1/1
  Constant3/1 -> Product3/2
  Constant2/1 -> Product2/2
  Delay2/1 -> Product3/1
  Product3/1 -> Sum1/2
  Sum1/1 -> Out2/1

== system fixed_point_model/Subsystem7/filter_with_comb2/Stage_1/Subsystem7 ==
  In2 : Inport
  Constant2 : Constant  Value=36
  Constant3 : Constant  Value=28
  Delay2 : Delay  DelayLength=1  InitialCondition=0  InputProcessing=Columns as channels (frame based)
  Product2 : Product
  Product3 : Product
  Sum1 : Sum  Inputs=|++
  Out2 : Outport
  wires:
  In2/1 -> Delay2/1, Product2/1
  Product2/1 -> Sum1/1
  Constant3/1 -> Product3/2
  Constant2/1 -> Product2/2
  Delay2/1 -> Product3/1
  Product3/1 -> Sum1/2
  Sum1/1 -> Out2/1

== system fixed_point_model/Subsystem7/filter_with_comb2/stage_3/Subsystem ==
  In1 : Inport
  Constant : Constant  Value=0.0006
  Constant1 : Constant  Value=-0.0051
  Constant2 : Constant  Value=0.0222
  Constant3 : Constant  Value=-0.0735
  Constant4 : Constant  Value=0.3058
  Constant5 : Constant  Value=0.3058
  Constant6 : Constant  Value=-0.0735
  Constant7 : Constant  Value=0.0222
  Constant8 : Constant  Value=-0.0051
  Constant9 : Constant  Value=0.0006
  Delay{1..9} (9 alike) : Delay  DelayLength=1  InitialCondition=0  InputProcessing=Columns as channels (frame based)
  Product{,1..9} (10 alike) : Product
  Sum : Sum  Inputs=|++++++++++
  Out1 : Outport
  wires:
  Product/1 -> Sum/1
  Product2/1 -> Sum/3
  Delay3/1 -> Product1/1, Delay4/1
  Sum/1 -> Out1/1
  Delay4/1 -> Product2/1, Delay5/1
  Product3/1 -> Sum/4
  In1/1 -> Product/2, Delay3/1
  Constant2/1 -> Product2/2
  Constant3/1 -> Product3/2
  Constant/1 -> Product/1
  Product1/1 -> Sum/2
  Constant1/1 -> Product1/2
  Delay5/1 -> Delay8/1, Product3/1
  Constant7/1 -> Product7/2
  Constant5/1 -> Product5/2
  Constant4/1 -> Product4/1
  Delay6/1 -> Product7/1, Delay9/1
  Delay2/1 -> Delay6/1, Product6/1
  Delay1/1 -> Delay2/1, Product5/1
  Constant6/1 -> Product6/2
  Constant8/1 -> Product8/2
  Constant9/1 -> Product9/2
  Delay7/1 -> Product9/1
  Product5/1 -> Sum/5
  Product6/1 -> Sum/6
  Product7/1 -> Sum/7
  Product8/1 -> Sum/8
  Product9/1 -> Sum/9
  Product4/1 -> Sum/10
  Delay8/1 -> Product4/2, Delay1/1
  Delay9/1 -> Product8/1, Delay7/1

== system fixed_point_model/Subsystem7/filter_with_comb2/stage_4/Subsystem1 ==
  Q' : Inport
  Constant : Constant  Value=-0.0012
  Constant1 : Constant  Value=0.0033
  Constant10 : Constant  Value=-0.0275
  Constant11 : Constant  Value=-0.0970
  Constant12 : Constant  Value=0.0150
  Constant13 : Constant  Value=-0.0076
  Constant14 : Constant  Value=0.0033
  Constant15 : Constant  Value=-0.0012
  Constant2 : Constant  Value=-0.0076
  Constant3 : Constant  Value=-0.0275
  Constant4 : Constant  Value=0.0495
  Constant5 : Constant  Value=0.0150
  Constant6 : Constant  Value=-0.0970
  Constant7 : Constant  Value=0.3152
  Constant8 : Constant  Value=0.3152
  Constant9 : Constant  Value=0.0495
  Delay{,1..14} (15 alike) : Delay  DelayLength=1  InitialCondition=0  InputProcessing=Columns as channels (frame based)
  Product{,1..15} (16 alike) : Product
  Sum : Sum  Inputs=|++++++++++++++++
  Out2 : Outport
  wires:
  Constant1/1 -> Product1/2
  Delay2/1 -> Delay3/1, Product4/1
  Constant10/1 -> Product11/2
  Constant9/1 -> Product10/2
  Delay/1 -> Delay1/1, Product1/1
  Delay4/1 -> Delay5/1, Product7/1
  Constant3/1 -> Product4/2
  Product8/1 -> Sum/11
  Product6/1 -> Sum/6
  Delay1/1 -> Product2/1, Delay14/1
  Delay5/1 -> Delay12/1, Product8/1
  Constant8/1 -> Product8/2
  Q'/1 -> Delay/1, Product/2
  Delay6/1 -> Delay7/1, Product10/1
  Constant/1 -> Product/1
  Constant11/1 -> Product9/2
  Product10/1 -> Sum/9
  Delay7/1 -> Delay8/1, Product11/1
  Product9/1 -> Sum/8
  Delay3/1 -> Product5/1, Delay13/1
  Constant4/1 -> Product5/2
  Product3/1 -> Sum/3
  Product5/1 -> Sum/5
  Constant2/1 -> Product2/2
  Constant5/1 -> Product3/2
  Constant7/1 -> Product7/2
  Product11/1 -> Sum/10
  Constant6/1 -> Product6/1
  Product/1 -> Sum/1
  Product1/1 -> Sum/2
  Product7/1 -> Sum/7
  Product4/1 -> Sum/4
  Sum/1 -> Out2/1
  Product2/1 -> Sum/12
  Constant12/1 -> Product12/2
  Delay8/1 -> Product12/1, Delay9/1
  Constant13/1 -> Product13/2
  Delay9/1 -> Delay10/1, Product13/1
  Constant14/1 -> Product14/2
  Delay10/1 -> Delay11/1, Product14/1
  Delay11/1 -> Product15/1
  Constant15/1 -> Product15/2
  Product12/1 -> Sum/13
  Product13/1 -> Sum/14
  Product14/1 -> Sum/15
  Product15/1 -> Sum/16
  Delay12/1 -> Delay6/1, Product9/1
  Delay13/1 -> Delay4/1, Product6/2
  Delay14/1 -> Delay2/1, Product3/1

== system fixed_point_model/Subsystem8/filter_with_comb1/Stage_1/Subsystem ==
  In1 : Inport
  Constant : Constant
  Constant1 : Constant  Value=42
  Constant2 : Constant  Value=21
  Delay1 : Delay  DelayLength=1  InitialCondition=0  InputProcessing=Columns as channels (frame based)
  Delay2 : Delay  DelayLength=1  InitialCondition=0  InputProcessing=Columns as channels (frame based)
  Product : Product
  Product1 : Product
  Product2 : Product
  Sum : Sum  Inputs=|+++
  Out1 : Outport
  wires:
  Constant1/1 -> Product1/2
  In1/1 -> Product/1, Delay1/1
  Product1/1 -> Sum/2
  Product/1 -> Sum/1
  Sum/1 -> Out1/1
  Constant/1 -> Product/2
  Delay1/1 -> Delay2/1, Product1/1
  Delay2/1 -> Product2/1
  Constant2/1 -> Product2/2
  Product2/1 -> Sum/3

== system fixed_point_model/Subsystem8/filter_with_comb1/Stage_1/Subsystem1 ==
  In2 : Inport
  Constant2 : Constant  Value=3
  Constant3 : Constant  Value=46
  Constant4 : Constant  Value=15
  Delay2 : Delay  DelayLength=1  InitialCondition=0  InputProcessing=Columns as channels (frame based)
  Delay3 : Delay  DelayLength=1  InitialCondition=0  InputProcessing=Columns as channels (frame based)
  Product2 : Product
  Product3 : Product
  Product4 : Product
  Sum1 : Sum  Inputs=|+++
  Out2 : Outport
  wires:
  Delay3/1 -> Product4/1
  Delay2/1 -> Delay3/1, Product3/1
  Sum1/1 -> Out2/1
  Constant2/1 -> Product2/2
  Product2/1 -> Sum1/1
  Constant3/1 -> Product3/2
  Product3/1 -> Sum1/2
  Constant4/1 -> Product4/2
  In2/1 -> Delay2/1, Product2/1
  Product4/1 -> Sum1/3

== system fixed_point_model/Subsystem8/filter_with_comb1/Stage_1/Subsystem2 ==
  In2 : Inport
  Constant2 : Constant  Value=6
  Constant3 : Constant  Value=48
  Constant4 : Constant  Value=10
  Delay2 : Delay  DelayLength=1  InitialCondition=0  InputProcessing=Columns as channels (frame based)
  Delay3 : Delay  DelayLength=1  InitialCondition=0  InputProcessing=Columns as channels (frame based)
  Product2 : Product
  Product3 : Product
  Product4 : Product
  Sum1 : Sum  Inputs=|+++
  Out2 : Outport
  wires:
  In2/1 -> Delay2/1, Product2/1
  Constant4/1 -> Product4/2
  Product2/1 -> Sum1/1
  Constant3/1 -> Product3/2
  Constant2/1 -> Product2/2
  Delay2/1 -> Delay3/1, Product3/1
  Product3/1 -> Sum1/2
  Sum1/1 -> Out2/1
  Delay3/1 -> Product4/1
  Product4/1 -> Sum1/3

== system fixed_point_model/Subsystem8/filter_with_comb1/Stage_1/Subsystem3 ==
  In2 : Inport
  Constant2 : Constant  Value=10
  Constant3 : Constant  Value=48
  Constant4 : Constant  Value=6
  Delay2 : Delay  DelayLength=1  InitialCondition=0  InputProcessing=Columns as channels (frame based)
  Delay3 : Delay  DelayLength=1  InitialCondition=0  InputProcessing=Columns as channels (frame based)
  Product2 : Product
  Product3 : Product
  Product4 : Product
  Sum1 : Sum  Inputs=|+++
  Out2 : Outport
  wires:
  In2/1 -> Delay2/1, Product2/1
  Constant4/1 -> Product4/2
  Product2/1 -> Sum1/1
  Constant3/1 -> Product3/2
  Constant2/1 -> Product2/2
  Delay2/1 -> Delay3/1, Product3/1
  Product3/1 -> Sum1/2
  Sum1/1 -> Out2/1
  Delay3/1 -> Product4/1
  Product4/1 -> Sum1/3

== system fixed_point_model/Subsystem8/filter_with_comb1/Stage_1/Subsystem4 ==
  In2 : Inport
  Constant2 : Constant  Value=15
  Constant3 : Constant  Value=46
  Constant4 : Constant  Value=3
  Delay2 : Delay  DelayLength=1  InitialCondition=0
  Delay3 : Delay  DelayLength=1  InitialCondition=0  InputProcessing=Columns as channels (frame based)
  Product2 : Product
  Product3 : Product
  Product4 : Product
  Sum1 : Sum  Inputs=|+++++
  Out2 : Outport
  wires:
  In2/1 -> Delay2/1, Product2/1
  Product4/1 -> Sum1/4
  Constant4/1 -> Product4/2
  Product2/1 -> Sum1/1
  Constant3/1 -> Product3/2
  Constant2/1 -> Product2/2
  Delay2/1 -> Delay3/1, Product3/1
  Product3/1 -> Sum1/2
  Sum1/1 -> Out2/1
  Delay3/1 -> Product4/1

== system fixed_point_model/Subsystem8/filter_with_comb1/Stage_1/Subsystem5 ==
  In2 : Inport
  Constant2 : Constant  Value=21
  Constant3 : Constant  Value=42
  Constant4 : Constant
  Delay2 : Delay  DelayLength=1  InitialCondition=0  InputProcessing=Columns as channels (frame based)
  Delay3 : Delay  DelayLength=1  InitialCondition=0  InputProcessing=Columns as channels (frame based)
  Product2 : Product
  Product3 : Product
  Product4 : Product
  Sum1 : Sum  Inputs=|+++
  Out2 : Outport
  wires:
  In2/1 -> Delay2/1, Product2/1
  Constant4/1 -> Product4/2
  Product2/1 -> Sum1/1
  Constant3/1 -> Product3/2
  Constant2/1 -> Product2/2
  Delay2/1 -> Delay3/1, Product3/1
  Product3/1 -> Sum1/2
  Sum1/1 -> Out2/1
  Delay3/1 -> Product4/1
  Product4/1 -> Sum1/3

== system fixed_point_model/Subsystem8/filter_with_comb1/Stage_1/Subsystem6 ==
  In2 : Inport
  Constant2 : Constant  Value=28
  Constant3 : Constant  Value=36
  Delay2 : Delay  DelayLength=1  InitialCondition=0  InputProcessing=Columns as channels (frame based)
  Product2 : Product
  Product3 : Product
  Sum1 : Sum  Inputs=|++
  Out2 : Outport
  wires:
  In2/1 -> Delay2/1, Product2/1
  Product2/1 -> Sum1/1
  Constant3/1 -> Product3/2
  Constant2/1 -> Product2/2
  Delay2/1 -> Product3/1
  Product3/1 -> Sum1/2
  Sum1/1 -> Out2/1

== system fixed_point_model/Subsystem8/filter_with_comb1/Stage_1/Subsystem7 ==
  In2 : Inport
  Constant2 : Constant  Value=36
  Constant3 : Constant  Value=28
  Delay2 : Delay  DelayLength=1  InitialCondition=0  InputProcessing=Columns as channels (frame based)
  Product2 : Product
  Product3 : Product
  Sum1 : Sum  Inputs=|++
  Out2 : Outport
  wires:
  In2/1 -> Delay2/1, Product2/1
  Product2/1 -> Sum1/1
  Constant3/1 -> Product3/2
  Constant2/1 -> Product2/2
  Delay2/1 -> Product3/1
  Product3/1 -> Sum1/2
  Sum1/1 -> Out2/1

== system fixed_point_model/Subsystem8/filter_with_comb1/stage_3/Subsystem ==
  In1 : Inport
  Constant : Constant  Value=0.0006
  Constant1 : Constant  Value=-0.0051
  Constant2 : Constant  Value=0.0222
  Constant3 : Constant  Value=-0.0735
  Constant4 : Constant  Value=0.3058
  Constant5 : Constant  Value=0.3058
  Constant6 : Constant  Value=-0.0735
  Constant7 : Constant  Value=0.0222
  Constant8 : Constant  Value=-0.0051
  Constant9 : Constant  Value=0.0006
  Delay{1..9} (9 alike) : Delay  DelayLength=1  InitialCondition=0  InputProcessing=Columns as channels (frame based)
  Product{,1..9} (10 alike) : Product
  Sum : Sum  Inputs=|++++++++++
  Out1 : Outport
  wires:
  Product/1 -> Sum/1
  Product2/1 -> Sum/3
  Delay3/1 -> Product1/1, Delay4/1
  Sum/1 -> Out1/1
  Delay4/1 -> Product2/1, Delay5/1
  Product3/1 -> Sum/4
  In1/1 -> Product/2, Delay3/1
  Constant2/1 -> Product2/2
  Constant3/1 -> Product3/2
  Constant/1 -> Product/1
  Product1/1 -> Sum/2
  Constant1/1 -> Product1/2
  Delay5/1 -> Delay8/1, Product3/1
  Constant7/1 -> Product7/2
  Constant5/1 -> Product5/2
  Constant4/1 -> Product4/1
  Delay6/1 -> Product7/1, Delay9/1
  Delay2/1 -> Delay6/1, Product6/1
  Delay1/1 -> Delay2/1, Product5/1
  Constant6/1 -> Product6/2
  Constant8/1 -> Product8/2
  Constant9/1 -> Product9/2
  Delay7/1 -> Product9/1
  Product5/1 -> Sum/5
  Product6/1 -> Sum/6
  Product7/1 -> Sum/7
  Product8/1 -> Sum/8
  Product9/1 -> Sum/9
  Product4/1 -> Sum/10
  Delay8/1 -> Product4/2, Delay1/1
  Delay9/1 -> Product8/1, Delay7/1
